simulink model "aero2_hardware_cascade_offline"  (R2024b)
settings: Solver=ode1  StartTime=0.0  StopTime=60  FixedStep=0.002  RelTol=1e-3
model workspace (MAT data in the model file):
  Dq = 2.25
  Kaw = 20
  Kff = 1
  Ki = 1.84164606325
  Kp = 0.216370391856
  Kq = 2.25
  ReferenceRate = [0 0.002 0.004 0.006 0.008 0.01 0.012 0.014 0.016 0.018 0.02 0.022 ... (90003 elements, 30001x3)]
  Ts = 0.002
  U_h = timeseries
  U_h.Name = 'unnamed'
  U_h.DataInfo = tsdata.datametadata
  U_h.DataInfo.Interpolation = tsdata.interpolation
  U_h.DataInfo.Interpolation.Fhandle : function handle (value not decoded)
  U_h.DataInfo.Interpolation.Name = 'linear'
  U_h.TimeInfo = tsdata.timemetadata
  U_h.TimeInfo.Length = 30001
  U_h.TimeInfo.DuplicateTimes = 0
  U_h.TimeInfo.Time_ = [0 0.002 0.004 0.006 0.008 0.01 0.012 0.014 0.016 0.018 0.02 0.022 ... (30001 elements, 30001x1)]
  U_h.TimeInfo.Initialized = 1
  U_h.QualityInfo = tsdata.qualmetadata
  U_h.Data_ = [0 0 0 0 0 0 0 0 0 0 0 0 ... (30001 elements, 30001x1)]
  U_v = timeseries
  U_v.Name = 'unnamed'
  U_v.DataInfo = tsdata.datametadata
  U_v.DataInfo.Interpolation = tsdata.interpolation
  U_v.DataInfo.Interpolation.Fhandle : function handle (value not decoded)
  U_v.DataInfo.Interpolation.Name = 'linear'
  U_v.TimeInfo = tsdata.timemetadata
  U_v.TimeInfo.Length = 30001
  U_v.TimeInfo.DuplicateTimes = 0
  U_v.TimeInfo.Time_ = [0 0.002 0.004 0.006 0.008 0.01 0.012 0.014 0.016 0.018 0.02 0.022 ... (30001 elements, 30001x1)]
  U_v.TimeInfo.Initialized = 1
  U_v.QualityInfo = tsdata.qualmetadata
  U_v.Data_ = [0 0 0 0 0 0 0 0 0 0 0 0 ... (30001 elements, 30001x1)]
  X0 = [0; 0; 0; 0]
  meas_on = 0
undefined symbols (not defined in the file): DiscIntNeverNeededParam
(part 1 of 2)
settings Model: Creator=matiasgarcia  LastModifiedBy=matiasgarcia
settings DebuggingCC: UnderspecifiedInitializationDetection=Classic  MergeDetectMultiDrivingBlocksExec=none  UnconnectedInputMsg=error  UnconnectedOutputMsg=error
settings ModelReferenceCC: PropagateSignalLabelsOutOfModel=off

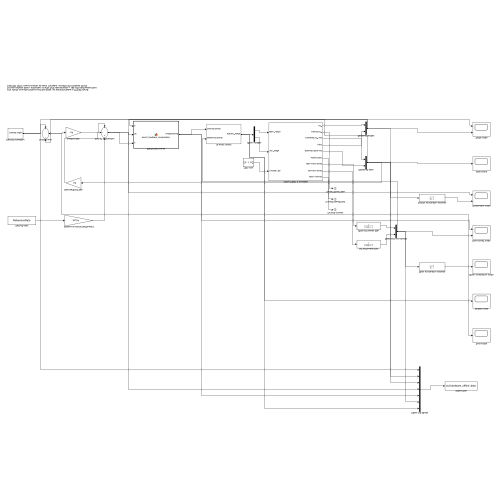
[thumbnail: Simulink's stored preview of the top-level diagram]
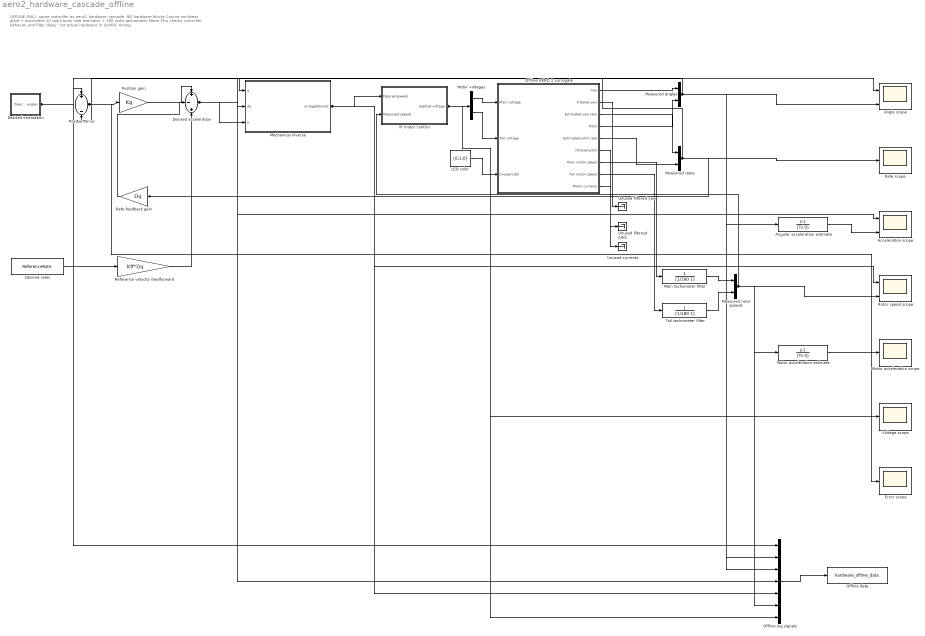
== system aero2_hardware_cascade_offline ==
  note: OFFLINE ONLY: same controller as aero2_hardware_cascade; NO hardware blocks
      | Course nonlinear plant + equivalent 10 rad/s body-rate estimator + 180 rad/s tachometer filters
      | This checks controller behavior and filter delay, not actual hardware or QUARC timing.
  Acceleration scope : Scope  NumInputPorts=2
  Angle scope : Scope  NumInputPorts=2
  Angular acceleration estimate : DiscreteTransferFcn  Numerator=[1 -1]  Denominator=[Ts 0]  SampleTime=Ts
  Desired acceleration : Sum  Inputs=+-+
  Desired orientation : Subsystem
  Desired rates : FromWorkspace  VariableName=ReferenceRate  OutputAfterFinalValue=Holding final value
  Error scope : Scope
  IP motor control : Subsystem
  LED color : Constant  Value=[0;1;0]
  Main tachometer filter : TransferFcn  Numerator=1  Denominator=[1/180 1]
  Measured angles : Mux  Inputs=2
  Measured rates : Mux  Inputs=2
  Measured rotor speeds : Mux  Inputs=2
  Mechanical inverse : MATLAB Function  TreatAsAtomicUnit=on
  Motor acceleration estimate : DiscreteTransferFcn  Numerator=[1 -1]  Denominator=[Ts 0]  SampleTime=Ts
  Motor acceleration scope : Scope
  Motor voltages : Demux  Outputs=2
  Offline AERO 2 surrogate : Subsystem
  Offline data : ToWorkspace  VariableName=hardware_offline_data  SaveFormat=Timeseries  SampleTime=-1
  Offline log signals : Mux  Inputs=7
  Position error : Sum  Inputs=+-
  Position gain : Gain  Gain=Kq
  Rate feedback gain : Gain  Gain=Dq
  Rate scope : Scope
  Reference velocity feedforward : Gain  Gain=Kff*Dq
  Rotor speed scope : Scope  NumInputPorts=2
  Tail tachometer filter : TransferFcn  Numerator=1  Denominator=[1/180 1]
  Unused currents : Terminator
  Unused filtered pitch : Terminator
  Unused filtered yaw : Terminator
  Voltage scope : Scope
  wires:
  Desired orientation/1(Desired angles) -> Position error/1, Angle scope/1, Offline log signals/1
  Measured angles/1 -> Position error/2, Mechanical inverse/1(q), Angle scope/2, Offline log signals/2
  Position error/1 -> Position gain/1, Error scope/1
  Position gain/1 -> Desired acceleration/1
  Measured rates/1 -> Rate feedback gain/1, Mechanical inverse/2(dq), Rate scope/1, Angular acceleration estimate/1, Offline log signals/3
  Rate feedback gain/1 -> Desired acceleration/2
  Desired rates/1 -> Reference velocity feedforward/1
  Reference velocity feedforward/1 -> Desired acceleration/3
  Desired acceleration/1 -> Mechanical inverse/3(a), Acceleration scope/1, Offline log signals/4
  Mechanical inverse/1(omegaDesired) -> IP motor control/1(Desired speeds), Rotor speed scope/1, Offline log signals/5
  Measured rotor speeds/1 -> IP motor control/2(Measured speeds), Rotor speed scope/2, Motor acceleration estimate/1, Offline log signals/6
  IP motor control/1(Applied voltage) -> Motor voltages/1, Voltage scope/1, Offline log signals/7
  Motor voltages/1 -> Offline AERO 2 surrogate/1(Main voltage)
  Motor voltages/2 -> Offline AERO 2 surrogate/2(Tail voltage)
  LED color/1 -> Offline AERO 2 surrogate/3(Unused LED)
  Offline AERO 2 surrogate/1(Yaw) -> Measured angles/1
  Offline AERO 2 surrogate/4(Pitch) -> Measured angles/2
  Offline AERO 2 surrogate/3(Estimated yaw rate) -> Measured rates/1
  Offline AERO 2 surrogate/5(Estimated pitch rate) -> Measured rates/2
  Offline AERO 2 surrogate/7(Main motor speed) -> Main tachometer filter/1
  Offline AERO 2 surrogate/8(Tail motor speed) -> Tail tachometer filter/1
  Main tachometer filter/1 -> Measured rotor speeds/1
  Tail tachometer filter/1 -> Measured rotor speeds/2
  Offline AERO 2 surrogate/2(Filtered yaw) -> Unused filtered yaw/1
  Offline AERO 2 surrogate/6(Filtered pitch) -> Unused filtered pitch/1
  Offline AERO 2 surrogate/9(Motor currents) -> Unused currents/1
  Angular acceleration estimate/1 -> Acceleration scope/2
  Motor acceleration estimate/1 -> Motor acceleration scope/1
  Offline log signals/1 -> Offline data/1
